simulink model "velocidad"  (R2018a)
settings: Solver=VariableStepAuto  StartTime=0.0  StopTime=30  RelTol=1e-3
undefined symbols (not defined in the file): a, b, c, d, f
settings Model: Creator=Karel  LastModifiedBy=Karel

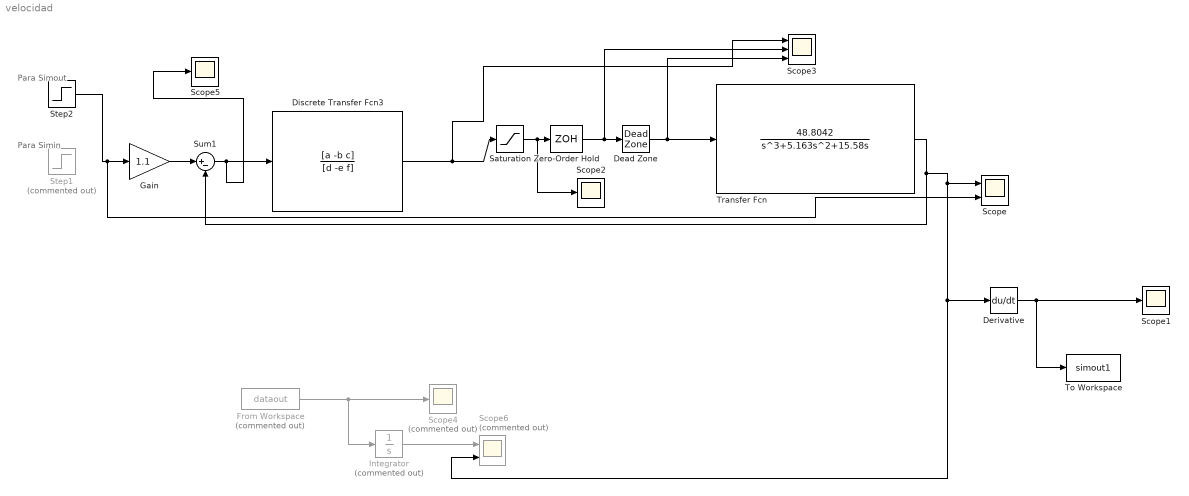
== system velocidad ==
  note: Para
      | Simout
  note: Para
      | Simin
  Dead Zone : DeadZone  LowerValue=0  UpperValue=0.2  SaturateOnIntegerOverflow=on
  Derivative : Derivative
  Discrete Transfer Fcn3 : DiscreteTransferFcn  Numerator=[a -b c]  Denominator=[d -e f]  SampleTime=27e-03
  From Workspace : FromWorkspace  Commented=on  VariableName=dataout  SampleTime=1e-2
  Gain : Gain  Gain=1.1
  Integrator : Integrator  Commented=on
  Saturation : Saturate  UpperLimit=10  LowerLimit=0
  Scope : Scope  NumInputPorts=2
  Scope1 : Scope
  Scope2 : Scope
  Scope3 : Scope  NumInputPorts=3
  Scope4 : Scope  Commented=on
  Scope5 : Scope
  Scope6 : Scope  Commented=on  NumInputPorts=2
  Step1 : Step  Commented=on  Time=8.8  After=12  SampleTime=0
  Step2 : Step  Time=8.4  After=9.89  SampleTime=0
  Sum1 : Sum  Inputs=|+-
  To Workspace : ToWorkspace  VariableName=simout1  SaveFormat=Structure With Time  SampleTime=-1
  Transfer Fcn : TransferFcn  Numerator=[48.8042]  Denominator=[1 5.163 15.58 0]
  Zero-Order Hold : ZeroOrderHold  SampleTime=-1
  wires:
  Gain/1 -> Sum1/1
  Dead Zone/1 -> Transfer Fcn/1, Scope3/3
  Sum1/1 -> Discrete Transfer Fcn3/1, Scope5/1
  Transfer Fcn/1 -> Scope6/2, Derivative/1, Scope/1, Sum1/2
  Discrete Transfer Fcn3/1 -> Saturation/1, Scope3/1
  Saturation/1 -> Scope2/1, Zero-Order Hold/1
  Zero-Order Hold/1 -> Scope3/2, Dead Zone/1
  Derivative/1 -> To Workspace/1, Scope1/1
  From Workspace/1 -> Integrator/1, Scope4/1
  Integrator/1 -> Scope6/1
  Step2/1 -> Scope/2, Gain/1
